simulink model "QDSWIRUpconversionSpectrometer"  (R2026a)
settings: Solver=FixedStepDiscrete  StartTime=0  StopTime=0  FixedStep=1
InitFcn:
  | qdPackageRoot=fileparts(fileparts(get_param(bdroot,'FileName')));addpath(qdPackageRoot);setupQDVoltageSelectedDualConverter();initQDSWIRUpconversionSpectrometer(false);clear qdPackageRoot;
undefined symbols (not defined in the file): qdCCDdarkElectrons, qdCCDNoiseElectrons, qdIncidentSpectrum, qdSpectrometerConfig, qdSpectrometerResponse
Description:
  | Bias-tuned CQD photodiode/QLED wavelength converter, visible CCD, and nonnegative spectral reconstruction
settings Model: Creator=jyohtiprakash  LastModifiedBy=jyohtiprakash

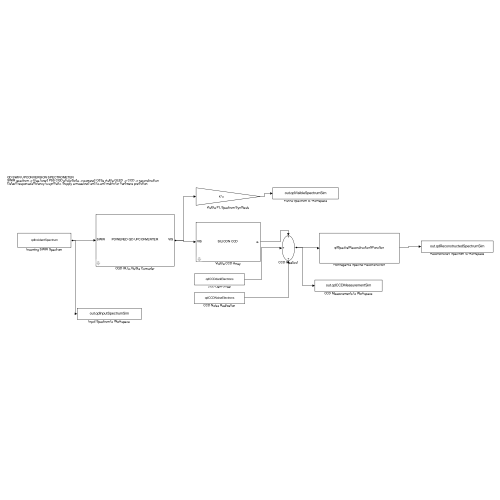
[thumbnail: Simulink's stored preview of the top-level diagram]
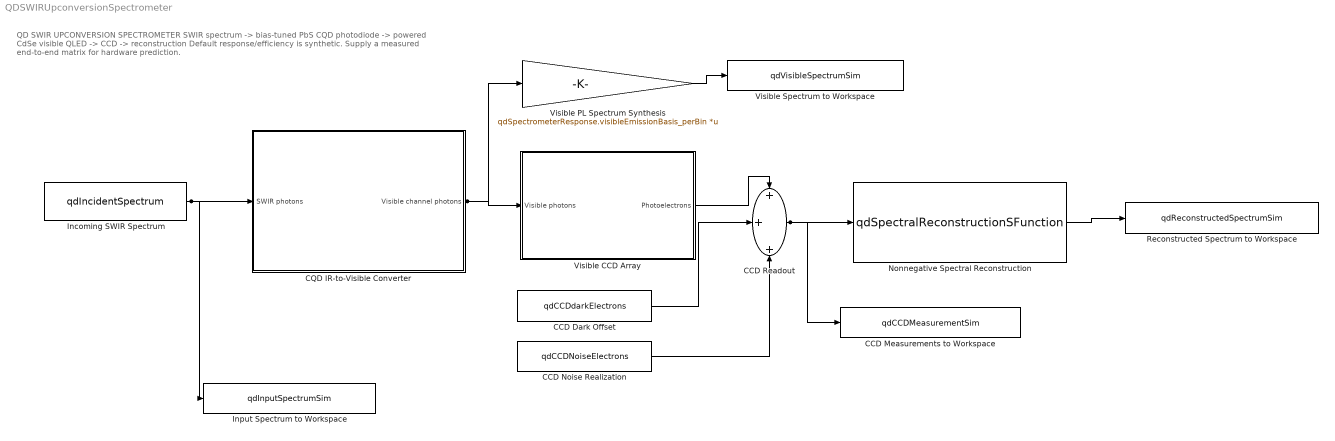
== system QDSWIRUpconversionSpectrometer ==
  note: QD SWIR UPCONVERSION SPECTROMETER
      | SWIR spectrum -> bias-tuned PbS CQD photodiode -> powered CdSe visible QLED -> CCD -> reconstruction
      | Default response/efficiency is synthetic. Supply a measured end-to-end matrix for hardware prediction.
  CCD Dark Offset : Constant  Value=qdCCDdarkElectrons
  CCD Measurements to Workspace : ToWorkspace  VariableName=qdCCDMeasurementSim  SaveFormat=Structure With Time  SampleTime=-1
  CCD Noise Realization : Constant  Value=qdCCDNoiseElectrons
  CCD Readout : Sum  Inputs=+++
  CQD IR-to-Visible Converter : Subsystem
      mask help: Small-bandgap PbS CQD sensitizer/photodiode driving a visible CdSe/ZnS QD emitter. Bias supplies the anti-Stokes energy.
      mask Display:
      | disp('POWERED QD UPCONVERTER');
      | port_label('input',1,'SWIR');
      | port_label('output',1,'VIS');
  Incoming SWIR Spectrum : Constant  Value=qdIncidentSpectrum
  Input Spectrum to Workspace : ToWorkspace  VariableName=qdInputSpectrumSim  SaveFormat=Structure With Time  SampleTime=-1
  Nonnegative Spectral Reconstruction : M-S-Function  FunctionName=qdSpectralReconstructionSFunction
  Reconstructed Spectrum to Workspace : ToWorkspace  VariableName=qdReconstructedSpectrumSim  SaveFormat=Structure With Time  SampleTime=-1
  Visible CCD Array : Subsystem
      mask help: Monochrome silicon CCD quantum efficiency, optical throughput, and pixel fill factor.
      mask Display:
      | disp('SILICON CCD');
      | port_label('input',1,'VIS');
      | port_label('output',1,'e-');
  Visible PL Spectrum Synthesis : Gain  Gain=qdSpectrometerResponse.visibleEmissionBasis_perBin  Multiplication=Matrix(K*u)
  Visible Spectrum to Workspace : ToWorkspace  VariableName=qdVisibleSpectrumSim  SaveFormat=Structure With Time  SampleTime=-1
  wires:
  Incoming SWIR Spectrum/1 -> CQD IR-to-Visible Converter/1(SWIR photons), Input Spectrum to Workspace/1
  CQD IR-to-Visible Converter/1(Visible channel photons) -> Visible PL Spectrum Synthesis/1, Visible CCD Array/1(Visible photons)
  Visible CCD Array/1(Photoelectrons) -> CCD Readout/1
  CCD Dark Offset/1 -> CCD Readout/2
  CCD Noise Realization/1 -> CCD Readout/3
  CCD Readout/1 -> Nonnegative Spectral Reconstruction/1, CCD Measurements to Workspace/1
  Visible PL Spectrum Synthesis/1 -> Visible Spectrum to Workspace/1
  Nonnegative Spectral Reconstruction/1 -> Reconstructed Spectrum to Workspace/1

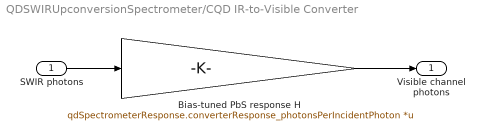
== system QDSWIRUpconversionSpectrometer/CQD IR-to-Visible Converter ==
  SWIR photons : Inport  PortDimensions=numel(qdSpectrometerConfig.inputWavelength_nm)
  Bias-tuned PbS response H : Gain  Gain=qdSpectrometerResponse.converterResponse_photonsPerIncidentPhoton  Multiplication=Matrix(K*u)
  Visible channel photons : Outport  PortDimensions=qdSpectrometerConfig.measurementCount
  wires:
  SWIR photons/1 -> Bias-tuned PbS response H/1
  Bias-tuned PbS response H/1 -> Visible channel photons/1

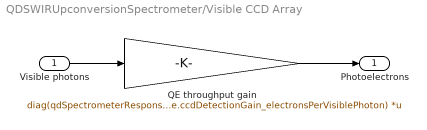
== system QDSWIRUpconversionSpectrometer/Visible CCD Array ==
  Visible photons : Inport  PortDimensions=qdSpectrometerConfig.measurementCount
  QE throughput gain : Gain  Gain=diag(qdSpectrometerResponse.ccdDetectionGain_electronsPerVisiblePhoton)  Multiplication=Matrix(K*u)
  Photoelectrons : Outport  PortDimensions=qdSpectrometerConfig.measurementCount
  wires:
  Visible photons/1 -> QE throughput gain/1
  QE throughput gain/1 -> Photoelectrons/1
